simulink model "Upravljac"  (R2025b)
settings: Solver=FixedStepAuto  StartTime=0.0  StopTime=3600  FixedStep=1  RelTol=1e-3
libraries: fuzblock x1
settings Model: Creator=trnav  LastModifiedBy=trnav

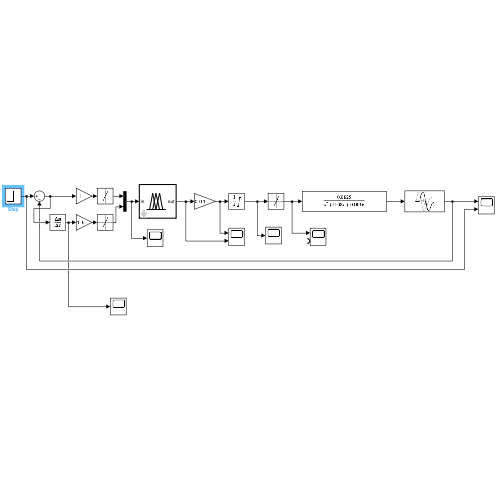
[thumbnail: Simulink's stored preview of the top-level diagram]
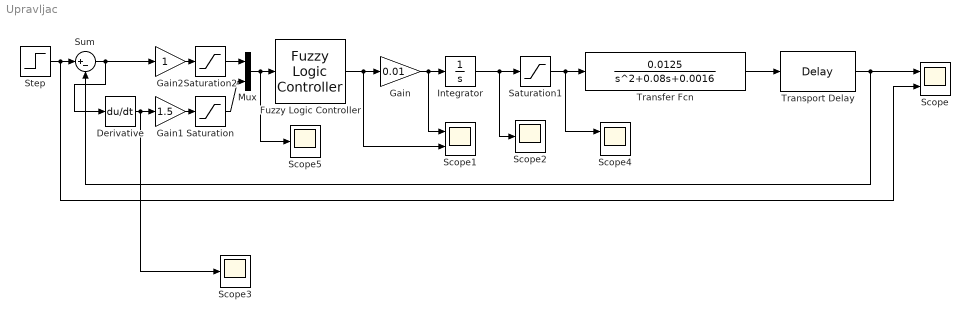
== system Upravljac ==
  Derivative : Derivative
  Fuzzy Logic Controller : fuzblock/Fuzzy Logic  Controller  FIS=fis  OutputSampleNumber=101  DataType=double  UseLookupTable=off  NumBreakpoints=10  FuzzifiedInputs=off  RuleFiringStrengths=off  RuleOutputs=off  AggregatedOutputs=off  SimulateUsing=Interpreted execution  OutOfRangeInputValueMessage=warning  NoRuleFiredMessage=warning  EmptyOutputFuzzySetMessage=warning
  Gain : Gain  Gain=0.01
  Gain1 : Gain  Gain=1.5
  Gain2 : Gain
  Integrator : Integrator  LimitOutput=on  UpperSaturationLimit=0.5  LowerSaturationLimit=-0.5
  Mux : Mux  Inputs=2
  Saturation : Saturate  UpperLimit=0.05  LowerLimit=-0.05
  Saturation1 : Saturate
  Saturation2 : Saturate  UpperLimit=2  LowerLimit=-2
  Scope : Scope  NumInputPorts=2
      settings: ActiveDisplayYMinimum=-3.6773885671895661  ActiveDisplayYMaximum=3.6764939248403419
  Scope1 : Scope  NumInputPorts=2
      settings: ActiveDisplayYMinimum=-0.11486513687600663  ActiveDisplayYMaximum=0.089767237593324389
  Scope2 : Scope
      settings: ActiveDisplayYMinimum=-1  ActiveDisplayYMaximum=1  DataLoggingVariableName=ScopeData2
  Scope3 : Scope
      settings: ActiveDisplayYMinimum=-0.073434221669424454  ActiveDisplayYMaximum=0.058820876847333586  DataLoggingVariableName=ScopeData3
  Scope4 : Scope  NumInputPorts=2
      settings: ActiveDisplayYMinimum=-0.44246560751031272  ActiveDisplayYMaximum=0.44558531813494906  DataLoggingVariableName=ScopeData4
  Scope5 : Scope
      settings: ActiveDisplayYMinimum=-2.5  ActiveDisplayYMaximum=2.5  DataLoggingVariableName=ScopeData5
  Step : Step  Time=1000  Before=-2  After=2  SampleTime=0
  Sum : Sum  Inputs=|+-
  Transfer Fcn : TransferFcn  Numerator=[0.0125]  Denominator=[1 0.08 0.0016]
  Transport Delay : TransportDelay  DelayTime=10
  wires:
  Transfer Fcn/1 -> Transport Delay/1
  Transport Delay/1 -> Scope/1, Sum/2
  Step/1 -> Scope/2, Sum/1
  Integrator/1 -> Saturation1/1, Scope2/1
  Saturation1/1 -> Scope4/1, Transfer Fcn/1
  Mux/1 -> Scope5/1, Fuzzy Logic Controller/1
  Saturation/1 -> Mux/2
  Saturation2/1 -> Mux/1
  Sum/1 -> Gain2/1, Derivative/1
  Fuzzy Logic Controller/1 -> Gain/1, Scope1/2
  Gain/1 -> Scope1/1, Integrator/1
  Gain1/1 -> Saturation/1
  Gain2/1 -> Saturation2/1
  Derivative/1 -> Scope3/1, Gain1/1
